simulink model "Aero_step_responses_pitch_from_yaw"  (R2025a)
settings: Solver=ode1  StartTime=0.0  StopTime=20  FixedStep=0.002  RelTol=1e-3  EnableMultiTasking=on
undefined symbols (not defined in the file or in its folder): HIL
libraries: quarc_library x3
settings Model: SimulationMode=external  ExtModeTrigDuration=5000  Creator=MLevis  LastModifiedBy=najem1u
settings SolverCC: AlgebraicLoopSolver=TrustRegion  PositivePriorityOrder=on
settings DataIOCC: LimitDataPoints=on  SaveFormat=Array  ReturnWorkspaceOutputs=off
settings DebuggingCC: SolverPrmCheckMsg=warning  UnconnectedInputMsg=warning  UnconnectedOutputMsg=warning  UnconnectedLineMsg=warning  SFUnexpectedBacktrackingDiag=warning  SFNoUnconditionalDefaultTransitionDiag=warning  SFExecutionAtInitializationDiag=none  ArithmeticOperatorsInVariantConditions=warning
settings ModelReferenceCC: PropagateSignalLabelsOutOfModel=off
settings SFSimCC: SimUseLocalCustomCode=off  CustomCodeUndefinedFunction=UseInterfaceOnly
settings RTWCC: SystemTargetFile=quarc_win64.tlc  TemplateMakefile=quarc_default_tmf  RTWUseLocalCustomCode=off  Toolchain=QUARC win64 | nmake (64-bit Windows)  BuildConfiguration=Faster Runs  GPUComputeCapability=3.5  Description=QUARC Win64 Target Using Toolchain
settings CodeAppCC: StateflowObjectComments=on
settings STFCustomTargetCC: SystemTargetFile=quarc_win64.tlc  MultiwordLength=2048.0  DynamicStringBufferSize=256.0  ConcurrentExecutionCompliant=on  UseToolchainInfoCompliant=on
settings GRTTargetCC: ExtMode=on  ExtModeMexFile=quarc_comm  TargetLangStandard=C89/C90 (ANSI)  ParMdlRefBuildCompliant=off  CompOptLevelCompliant=off  CombineOutputUpdateFcns=off  MatFileLogging=off  CPPClassGenCompliant=off  GRTInterface=on
settings ConfigComp: CovMetricSettings=dw  CovSaveCumulativeToWorkspaceVar=on  CovSaveSingleToWorkspaceVar=on  CovExternalEMLEnable=off  CovSFcnEnable=off

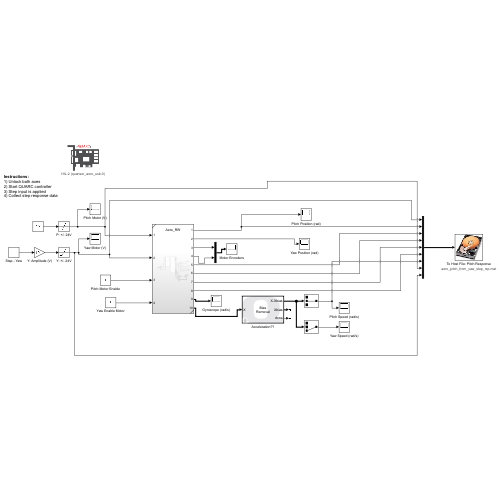
[thumbnail: Simulink's stored preview of the top-level diagram]
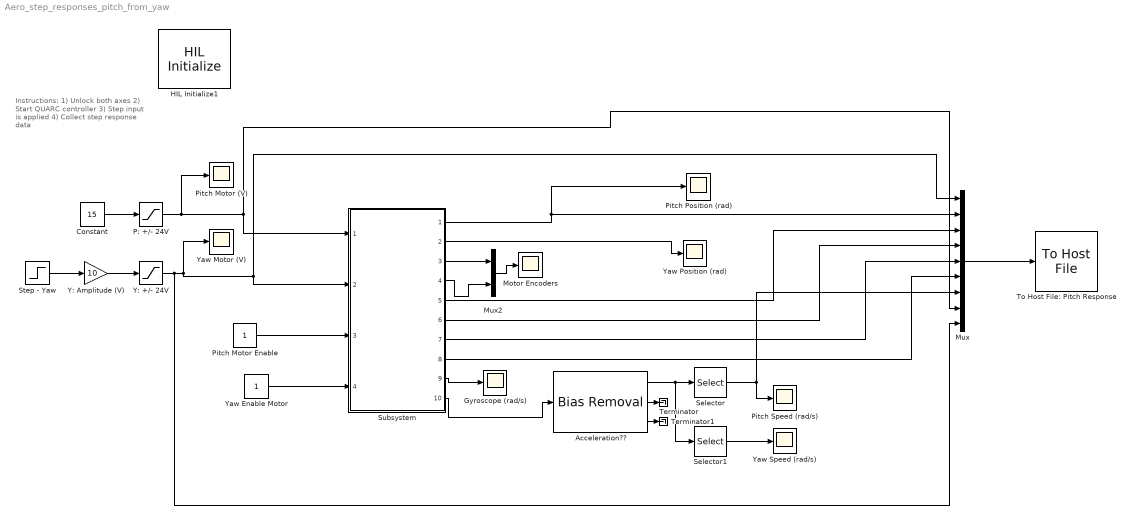
== system Aero_step_responses_pitch_from_yaw ==
  note: Instructions:
      | 1) Unlock both axes
      | 2) Start QUARC controller
      | 3) Step input is applied
      | 4) Collect step response data
  Acceleration?? : quarc_library/Discrete/Bias Removal  start_time=0  end_time=1  switch_id=0  sample_time=qc_get_step_size
      settings: SourceProductName=QUARC Targets
  Constant : Constant  Value=15
  Gyroscope (rad/s) : Scope
      settings: TimeSpan=10  ActiveDisplayYMinimum=-2  ActiveDisplayYMaximum=2  DataLoggingVariableName=ScopeData9  DataLoggingSaveFormat=Array
  HIL Initialize1 : quarc_library/Data Acquisition/Generic/Configuration/HIL Initialize  Priority=-99  object_name=HIL-2  board_type=quanser_aero_usb  board_number=0  board_options=""  exclusive=off  active=off  hardware_clocks=[0]  clock_modes=[]  initial_clock_frequencies=[]  set_clock_params_at_start=off  set_clock_params_at_switch_in=off  set_clock_frequencies_at_start=off  set_clock_frequencies_at_switch_in=off  analog_input_channels=[0:1]  analog_input_configurations=[]  analog_input_maximums=3  analog_input_minimums=-3  set_analog_input_params_at_start=off  set_analog_input_params_at_switch_in=off  analog_output_channels=[0:1]  analog_output_maximums=24  analog_output_minimums=-24  initial_analog_outputs=[0]  final_analog_outputs=[0]  watchdog_analog_outputs=[0]  set_analog_output_params_at_start=off  set_analog_output_params_at_switch_in=off  set_analog_outputs_at_start=on  set_analog_outputs_at_switch_in=off  set_analog_outputs_at_terminate=on  set_analog_outputs_at_switch_out=off  set_analog_outputs_on_watchdog=on  digital_input_channels=[]  digital_output_channels=[0:1]  digital_output_configuration=[]  initial_digital_outputs=[1]  final_digital_outputs=[0]  watchdog_digital_outputs=[0]  set_digital_output_params_at_start=off  set_digital_output_params_at_switch_in=off  set_digital_outputs_at_start=on  set_digital_outputs_at_switch_in=off  set_digital_outputs_at_terminate=on  set_digital_outputs_at_switch_out=off  set_digital_outputs_on_watchdog=on  encoder_channels=[0:3]  quadrature=[4]  encoder_filter_frequency=[]  initial_encoder_counts=[0]  set_encoder_params_at_start=off  set_encoder_params_at_switch_in=off  set_encoder_counts_at_start=on  set_encoder_counts_at_switch_in=off  pwm_channels=[]  pwm_modes=[]  pwm_frequency=[]  pwm_configuration=[]  pwm_alignment=[]  pwm_polarity=[]  pwm_leading_deadband=[]  pwm_trailing_deadband=[]  initial_pwm_outputs=[]  final_pwm_outputs=[]  watchdog_pwm_outputs=[]  set_pwm_params_at_start=off  set_pwm_params_at_switch_in=off  set_pwm_outputs_at_start=off  set_pwm_outputs_at_switch_in=off  set_pwm_outputs_at_terminate=off  set_pwm_outputs_at_switch_out=off  set_pwm_outputs_on_watchdog=off  other_output_channels=[11000:11002]  initial_other_outputs=[0 1 0]  final_other_outputs=[1 0 0]  watchdog_other_outputs=[0 0 1]  set_other_outputs_at_start=on  set_other_outputs_at_switch_in=off  set_other_outputs_at_terminate=on  set_other_outputs_at_switch_out=off  set_other_outputs_on_watchdog=on
  Motor Encoders : Scope
      settings: ActiveDisplayYMinimum=-500000  ActiveDisplayYMaximum=0  DataLoggingSaveFormat=Array
  Mux : Mux  Inputs=9
  Mux2 : Mux  Inputs=2
  P: +/- 24V : Saturate  UpperLimit=24  LowerLimit=-24
  Pitch Motor (V) : Scope
      settings: TimeSpan=5  ActiveDisplayYMinimum=-25  ActiveDisplayYMaximum=25  DataLoggingVariableName=ScopeData2  DataLoggingSaveFormat=Array
  Pitch Motor Enable : Constant
  Pitch Position (rad) : Scope
      settings: TimeSpan=5  ActiveDisplayYMinimum=-1.5  ActiveDisplayYMaximum=1.5  DataLoggingVariableName=ScopeData3  DataLoggingSaveFormat=Array
  Pitch Speed (rad/s) : Scope
      settings: TimeSpan=5  ActiveDisplayYMinimum=-1.5  ActiveDisplayYMaximum=1.5  DataLoggingVariableName=pitch_spd  DataLoggingSaveFormat=Array
  Selector : Selector  InputPortWidth=3  IndexOptions=Index vector (dialog)  Indices=[2]  OutputSizes=1
  Selector1 : Selector  InputPortWidth=3  IndexOptions=Index vector (dialog)  Indices=[3]  OutputSizes=1
  Step - Yaw : Step  Time=2  SampleTime=0
  Subsystem : Subsystem  ReferencedSubsystem=Aero_RW
  Terminator : Terminator
  Terminator1 : Terminator
  To Host File: Pitch Response : quarc_library/Sinks/To Host/To Host File  source=Specify via dialog (do not evaluate)  file_name=aero_pitch_from_yaw_step_rsp.mat  variable_name=step_rsp_py  decimation=1  sample_time=-1  file_format=MAT-file v.4  options=No header or footer  append=off  final_file_name=aero_pitch_from_yaw_step_rsp.mat  encoding=Default  bitrate=0
  Y: +/- 24V : Saturate  UpperLimit=24  LowerLimit=-24
  Y: Amplitude (V) : Gain  Gain=10
  Yaw Enable Motor : Constant
  Yaw Motor (V) : Scope
      settings: TimeSpan=5  ActiveDisplayYMinimum=-25  ActiveDisplayYMaximum=25  DataLoggingVariableName=ScopeData5  DataLoggingSaveFormat=Array
  Yaw Position (rad) : Scope
      settings: TimeSpan=5  ActiveDisplayYMinimum=-0.5  ActiveDisplayYMaximum=1.5  DataLoggingVariableName=ScopeData4  DataLoggingSaveFormat=Array
  Yaw Speed (rad/s) : Scope
      settings: TimeSpan=5  ActiveDisplayYMinimum=-0.5  ActiveDisplayYMaximum=1.5  DataLoggingVariableName=pitch_spd1  DataLoggingSaveFormat=Array
  wires:
  P: +/- 24V/1 -> Mux/8, Subsystem/1, Pitch Motor (V)/1
  Constant/1 -> P: +/- 24V/1
  Subsystem/2 -> Yaw Position (rad)/1
  Mux/1 -> To Host File: Pitch Response/1
  Acceleration??/2 -> Terminator/1
  Acceleration??/3 -> Terminator1/1
  Acceleration??/1 -> Selector1/1, Selector/1
  Selector/1 -> Mux/7, Pitch Speed (rad/s)/1
  Step - Yaw/1 -> Y: Amplitude (V)/1
  Y: Amplitude (V)/1 -> Y: +/- 24V/1
  Selector1/1 -> Yaw Speed (rad/s)/1
  Y: +/- 24V/1 -> Mux/9, Mux/1, Subsystem/2, Yaw Motor (V)/1
  Pitch Motor Enable/1 -> Subsystem/3
  Yaw Enable Motor/1 -> Subsystem/4
  Subsystem/9 -> Gyroscope (rad/s)/1
  Subsystem/10 -> Acceleration??/1
  Mux2/1 -> Motor Encoders/1
  Subsystem/3 -> Mux2/1
  Subsystem/4 -> Mux2/2
  Subsystem/1 -> Pitch Position (rad)/1, Mux/2
  Subsystem/6 -> Mux/4
  Subsystem/7 -> Mux/5
  Subsystem/5 -> Mux/3
  Subsystem/8 -> Mux/6
